simulink model "f01_spring"  (R2024b)
settings: Solver=FixedStepDiscrete  StartTime=0.0  StopTime=4  FixedStep=0.2  RelTol=1e-3
model workspace (MAT data in the model file):
  S02_Ad = [0.962300258554  0.182366876725; -0.36473375345  0.816406757174]
  S02_Ad11 = 0.962300258554
  S02_Ad12 = 0.182366876725
  S02_Ad21 = -0.36473375345
  S02_Ad22 = 0.816406757174
  S02_Bd = [0.0188498707231; 0.182366876725]
  S02_Bd1 = 0.0188498707231
  S02_Bd2 = 0.182366876725
  S02_C = [1 0]
  S02_dt = 0.2
  S02_input_gain = 1
  S02_x0 = [0.1; -0.05]
  S02_x01 = 0.1
  S02_x02 = -0.05
settings Model: Creator=sk3547969879  LastModifiedBy=sk3547969879

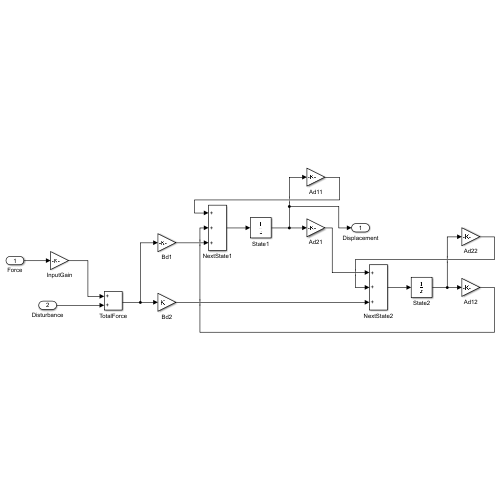
[thumbnail: Simulink's stored preview of the top-level diagram]
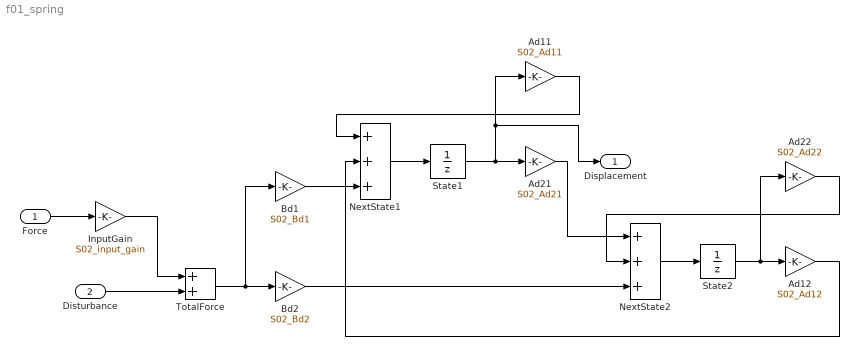
== system f01_spring ==
  Force : Inport
  Disturbance : Inport  Port=2
  Ad11 : Gain  Gain=S02_Ad11
  Ad12 : Gain  Gain=S02_Ad12
  Ad21 : Gain  Gain=S02_Ad21
  Ad22 : Gain  Gain=S02_Ad22
  Bd1 : Gain  Gain=S02_Bd1
  Bd2 : Gain  Gain=S02_Bd2
  InputGain : Gain  Gain=S02_input_gain
  NextState1 : Sum  Inputs=+++
  NextState2 : Sum  Inputs=+++
  State1 : UnitDelay  InitialCondition=S02_x01  SampleTime=S02_dt  HasFrameUpgradeWarning=on
  State2 : UnitDelay  InitialCondition=S02_x02  SampleTime=S02_dt  HasFrameUpgradeWarning=on
  TotalForce : Sum
  Displacement : Outport
  wires:
  NextState2/1 -> State2/1
  Bd2/1 -> NextState2/3
  Ad22/1 -> NextState2/2
  Ad21/1 -> NextState2/1
  NextState1/1 -> State1/1
  Bd1/1 -> NextState1/3
  Ad12/1 -> NextState1/2
  Ad11/1 -> NextState1/1
  TotalForce/1 -> Bd1/1, Bd2/1
  State2/1 -> Ad12/1, Ad22/1
  State1/1 -> Ad11/1, Displacement/1, Ad21/1
  Disturbance/1 -> TotalForce/2
  InputGain/1 -> TotalForce/1
  Force/1 -> InputGain/1
